simulink model "sf_temporal_logic_from_junction"  (R2025b)
settings: Solver=FixedStepDiscrete  StartTime=0.0  StopTime=30  FixedStep=1  RelTol=1e-3  EnableMultiTasking=on
settings Model: Creator=The MathWorks, Inc.  LastModifiedBy=The MathWorks, Inc.
settings SolverCC: AlgebraicLoopSolver=TrustRegion
settings DataIOCC: LimitDataPoints=on  SaveFormat=Array  ReturnWorkspaceOutputs=off
settings OptimizationCC: ReuseModelBlockBuffer=off  ExpressionDepthLimit=2147483647.0  LifeSpan=inf
settings DebuggingCC: UnderspecifiedInitializationDetection=Classic  MergeDetectMultiDrivingBlocksExec=none  SolverPrmCheckMsg=warning  FcnCallInpInsideContextMsg=warning  UnconnectedInputMsg=warning  UnconnectedOutputMsg=warning  UnconnectedLineMsg=warning  StateNameClashWarn=warning  SFUnexpectedBacktrackingDiag=warning  SFNoUnconditionalDefaultTransitionDiag=warning  SFExecutionAtInitializationDiag=none  ArithmeticOperatorsInVariantConditions=warning
settings HardwareCC: ProdBitPerPointer=32.0  ProdBitPerSizeT=32.0  ProdBitPerPtrDiffT=32.0  ProdLargestAtomicFloat=None  ProdIntDivRoundTo=Undefined  ProdEndianess=Unspecified  ProdWordSize=32.0  ProdHWDeviceType=32-bit Generic
settings ModelReferenceCC: EnableRefExpFcnMdlSchedulingChecks=on  PropagateSignalLabelsOutOfModel=off
settings SFSimCC: SimUseLocalCustomCode=off  SimParseCustomCode=off  CustomCodeUndefinedFunction=UseInterfaceOnly
settings RTWCC: RTWUseLocalCustomCode=off  GPUComputeCapability=3.5
settings CodeAppCC: StateflowObjectComments=on
settings GRTTargetCC: TargetLangStandard=C89/C90 (ANSI)  CombineOutputUpdateFcns=off  GRTInterface=on
settings ConfigComp: CovMetricSettings=dw  CovSaveCumulativeToWorkspaceVar=on  CovSaveSingleToWorkspaceVar=on  CovExternalEMLEnable=off

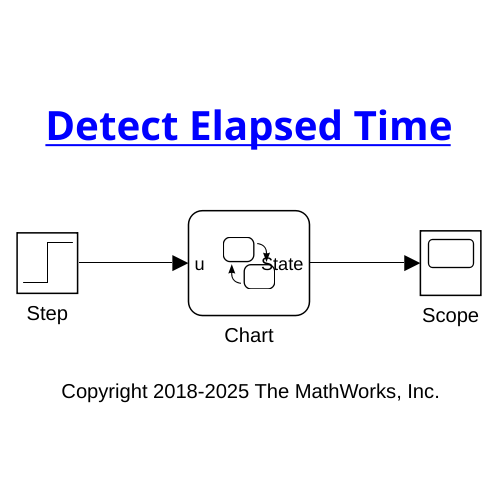
[thumbnail: Simulink's stored preview of the top-level diagram]
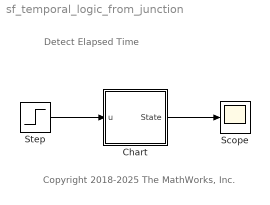
== system sf_temporal_logic_from_junction ==
  note: Copyright 2018-2025 The MathWorks, Inc.
  note: Detect Elapsed Time
  Chart : Stateflow chart  TreatAsAtomicUnit=on
  Scope : Scope
      settings: ActiveDisplayYMinimum=0.75  ActiveDisplayYMaximum=4.25
  Step : Step  Time=3  SampleTime=0
  wires:
  Step/1 -> Chart/1(u)
  Chart/1(State) -> Scope/1

== stateflow chart sf_temporal_logic_from_junction/Chart ==
  state Fast
  state Start
  state Medium
  state Slow
  (default) -> Start
  (junction 23) -> Fast : before(2,sec)
  (junction 4) -> (junction 23) [order 1]
  Start -> (junction 4) : [u == 1]
  (junction 4) -> Medium [order 3]
  (junction 4) -> (junction 26) [order 2]
  (junction 26) -> Slow : after(5,sec)
  data: u input; State output Enum: SlowMediumFast
